simulink model "canal_cbs"  (R2023b)
settings: Solver=VariableStepAuto  StartTime=0.0  StopTime=100  RelTol=1e-3
values from neighbouring files (symbols this model uses):
  graine = round(P.graine)    [Parametres.m]    (also in parametres_perso.m = mod(sum(c .* (1:numel(c)) * 31) + 7 * numel(c), 2^31 - 1))
  p1 = P.p1    [Parametres.m]
  pe = P.pe_cbs    [Parametres.m]
  Tb = 1    [Parametres.m]
settings Model: Creator=e2508348  LastModifiedBy=e2508348

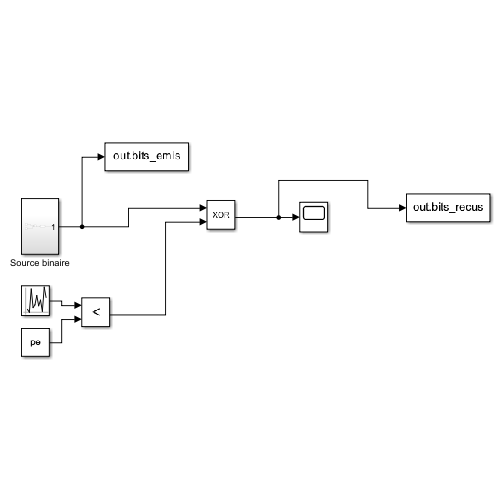
[thumbnail: Simulink's stored preview of the top-level diagram]
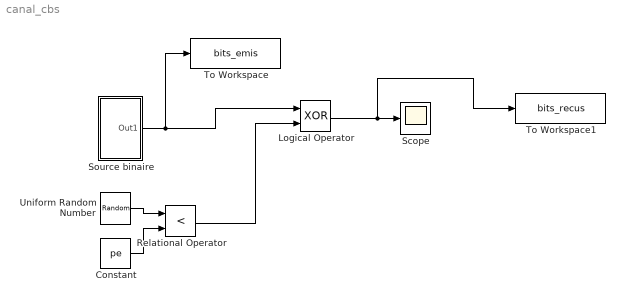
== system canal_cbs ==
  Constant : Constant  Value=pe
  Logical Operator : Logic  Operator=XOR  AllPortsSameDT=off  OutDataTypeStr=boolean
  Relational Operator : RelationalOperator  Operator=<  OutDataTypeStr=boolean  RndMeth=Simplest  InputSameDT=off
  Scope : Scope
  Source binaire : Subsystem
  To Workspace : ToWorkspace  VariableName=bits_emis  SampleTime=-1
  To Workspace1 : ToWorkspace  VariableName=bits_recus  SampleTime=-1
  Uniform Random Number : UniformRandomNumber  Minimum=0  Seed=graine+1  SampleTime=Tb
  wires:
  Uniform Random Number/1 -> Relational Operator/1
  Constant/1 -> Relational Operator/2
  Source binaire/1(Out1) -> To Workspace/1, Logical Operator/1
  Relational Operator/1 -> Logical Operator/2
  Logical Operator/1 -> To Workspace1/1, Scope/1

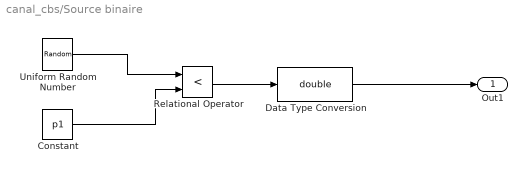
== system canal_cbs/Source binaire ==
  Constant : Constant  Value=p1
  Data Type Conversion : DataTypeConversion  OutDataTypeStr=double  SaturateOnIntegerOverflow=off  RndMeth=Floor
  Relational Operator : RelationalOperator  Operator=<  OutDataTypeStr=boolean  RndMeth=Simplest  InputSameDT=off
  Uniform Random Number : UniformRandomNumber  Minimum=0  Seed=graine  SampleTime=Tb
  Out1 : Outport
  wires:
  Data Type Conversion/1 -> Out1/1
  Relational Operator/1 -> Data Type Conversion/1
  Constant/1 -> Relational Operator/2
  Uniform Random Number/1 -> Relational Operator/1
